simulink model "RobustFormationControl_FractionalModel"  (R2023a)
settings: Solver=ode3  StartTime=0.0  StopTime=30  FixedStep=0.0001  RelTol=1e-3
InitFcn:
  | % close all;
  | % clear all;
  | % clc;
  | % System & Qaudrotor Parameters
  | %==============================
  | m = 0.486;                                         % Quadrotor Mass ( kg )
  | 
  | L = 0.25;                                         % Length of the arm ( m )
  | % L = 0.25;                                         % Length of the arm ( m )
  | 
  | Ixx = 4.856e-03; Iyy = 4.856e-03; Izz = 8.801e-03; % The moments of inertia around x,y and z axes respectively ( kg.m^2 )
  | % Ixx = 3.8278e-03; Iyy = 3.8278e-03; Izz = 7.6566e-03; % The moments of inertia around x,y and z axes respectively ( kg.m^2 )
  | 
  | Jr = 2.8385e-5;                                            % The inertia moment of rotor ( kg.m^2 )
  | % Jr = 0;
  | 
  | % Kx=5.5670e-4;
  | % Ky=5.5670e-4;
  | % Kz=6.3540e-4;
  | % kx=0.032;
  | % ky=0.032;
  | % kz=0.048;
  | Kfx = 5.5670e-4; Kfy = 5.5670e-4; Kfz = 6.3540e-4;% The Rotational drag cofficients ( N/rad/s )
  | 
  | % Ktx = 0.032; Kty = 0.032; Ktz = 0.048;               % The linear drag coefficients in x, y, z respectively ( N/m/s )
  | Ktx = 5.5670e-4; Kty =5.5670e-4; Ktz = 6.3540e-4;               % The linear drag coefficients in x, y, z respectively ( N/m/s )
  | 
  | b = 2.923e-05;                                      % The lift coefficient
  | % b = 2.9842e-05;                                      % The lift coefficient
  | 
  | d = 1.12e-06;                                       % The drag coefficient
  | % d = 3.2320e-07;                                       % The drag coefficient
  | 
  | g = 9.81;                                          % The acceleration due to gravity ( m/s^2 )
  | 
  | %-------- The Coefficients of Non-linear Equations of Quadrotor ( Page 11) -------
  | %--------------------------------------------------------------------------------
  | % Rotational Equations
  | %=====================
  | % Coefficients in ( eq1 ) >>..
  | a1 = (Iyy - Izz)/Ixx;
  | b1 = - Jr/Ixx;
  | c1 = - Kfx/Ixx;
  | d1 = L/Ixx;
  | 
  | % Coefficients in ( eq2 ) >>..
  | a2 = (Izz - Ixx)/Iyy;
  | b2 = Jr/Iyy;
  | c2 = - Kfy/Iyy;
  | d2 = L/Iyy;
  | 
  | % Coefficients in ( eq3 ) >>..
  | a3 = (Ixx - Iyy)/Izz;
  | b3 = - Kfz/Izz;
  | c3 = 1/Izz;
  | % c3 = d/Izz;
  | 
  | % Translational Equations
  | %========================
  | % Coefficients in ( eq4 ) >>..
  | ... (+151 lines)
libraries: fod x135, eeStairGenerator x5
(part 8 of 9)

== system RobustFormationControl_FractionalModel/Fractional Leader with four followers/Follower 3 System/Follower 2 Quadrotor Model/Control Module1/Subsystem6/Subsystem4 ==
  x8 : Inport
  xL : Inport  Port=2
  dX : Inport  Port=3
  Derivative{,1..3} (4 alike) : Derivative
  Divide2 : Product  Inputs=**  RndMeth=Zero  SaturateOnIntegerOverflow=on
  Gain1 : Gain  Commented=on  Gain=a6
  Sum : Sum  Inputs=-+-
  D1 : Outport
  wires:
  Sum/1 -> D1/1
  x8/1 -> Divide2/2
  Divide2/1 -> Sum/1
  [a4D] -> Divide2/1
  Derivative/1 -> Derivative1/1
  xL/1 -> Derivative/1
  Derivative3/1 -> Sum/3
  Derivative2/1 -> Derivative3/1
  dX/1 -> Derivative2/1
  Derivative1/1 -> Sum/2

== system RobustFormationControl_FractionalModel/Fractional Leader with four followers/Follower 3 System/Follower 2 Quadrotor Model/Control Module1/Subsystem6/Subsystem5 ==
  xL : Inport
  x7 : Inport  Port=2
  x8 : Inport  Port=3
  dX : Inport  Port=4
  S8 : Inport  Port=5
  Abs : Abs  SaturateOnIntegerOverflow=off
  Derivative : Derivative
  Derivative1 : Derivative
  Divide{,1..4} (5 alike) : Product  Inputs=**  RndMeth=Zero  SaturateOnIntegerOverflow=on
  Gain : Gain  Gain=q0
  Gain1 : Gain  Gain=q1
  Gain2 : Gain  Gain=q2
  Integrator : Integrator
  Integrator1 : Integrator
  Integrator2 : Integrator
  Sum2 : Sum  Inputs=++++
  Sum4 : Sum  Inputs=+--
  Sum5 : Sum  Inputs=+--
  Tanh : Trigonometry  Operator=tanh
  w : Constant  Value=w
  D3 : Outport  VectorParamsAs1DForOutWhenUnconnected=off
  wires:
  S8/1 -> [S8], Abs/1
  Gain/1 -> Integrator/1
  Integrator/1 -> Sum2/1  "B0"
  [e1] -> Divide/2
  Gain1/1 -> Integrator1/1
  Divide/1 -> Gain1/1
  Divide1/1 -> Gain2/1
  Gain2/1 -> Integrator2/1
  [e2] -> Divide1/2
  Abs/1 -> Divide1/1, Divide/1, Gain/1
  Integrator1/1 -> Divide3/2  "B1"
  w/1 -> Sum2/4
  Tanh/1 -> Divide2/2
  [S8] -> Tanh/1
  Divide2/1 -> D3/1
  [e1] -> Divide3/1
  [e2] -> Divide4/1
  Integrator2/1 -> Divide4/2  "B2"
  Divide3/1 -> Sum2/2
  Divide4/1 -> Sum2/3
  Sum2/1 -> Divide2/1
  Derivative1/1 -> Sum4/3
  Derivative/1 -> Sum4/1
  Sum4/1 -> [e2]
  Sum5/1 -> [e1]
  xL/1 -> Sum5/1, Derivative/1
  x8/1 -> Sum4/2
  dX/1 -> Sum5/3, Derivative1/1
  x7/1 -> Sum5/2

== system RobustFormationControl_FractionalModel/Fractional Leader with four followers/Follower 3 System/Follower 2 Quadrotor Model/Control Module1/Subsystem8/Subsystem ==
  x3 : Inport
  xd3 : Inport  Port=2
  x4 : Inport  Port=3
  xd4 : Inport  Port=4
  S4 : Inport  Port=5
  Constant : Constant  Value=p/q
  Constant1 : Constant  Value=gammaP(2)-1
  Divide : Product  Inputs=**  RndMeth=Zero  SaturateOnIntegerOverflow=on
  Fractional derivative : fod/Fractional derivative  gam=alpha1(2)  ww=[0.001; 1000]  n=5  nFod=off
      settings: SourceProductName=FOMCON Toolbox
  Fractional integrator1 : fod/Fractional integrator  gam=alpha2(2)  ww=[0.001; 1000]  n=5  nFod=off
      settings: SourceProductName=FOMCON Toolbox
  Gain : Gain  Gain=cTheta1
  Gain1 : Gain  Gain=cTheta2
  Gain2 : Gain  Gain=gammaP(2)
  Gain3 : Gain  Gain=Sigma1Theta
  Gain4 : Gain  Gain=Sigma2Theta
  Power : Math  Operator=pow
  Power1 : Math  Operator=pow
  Sum : Sum
  Sum1 : Sum  Inputs=+-
  Sum2 : Sum  Inputs=---
  Sum3 : Sum  Inputs=+-
  Tanh : Trigonometry  Operator=tanh
  D2 : Outport  VectorParamsAs1DForOutWhenUnconnected=off
  wires:
  xd4/1 -> Sum1/2
  xd3/1 -> Sum3/2
  x3/1 -> Sum3/1
  x4/1 -> Sum1/1
  Sum3/1 -> Power1/1, Power/1
  Constant/1 -> Power/2
  Power/1 -> Gain/1
  Gain/1 -> Fractional derivative/1
  Constant1/1 -> Power1/2
  Power1/1 -> Divide/2
  Divide/1 -> Gain1/1
  Gain1/1 -> Gain2/1
  Sum1/1 -> Divide/1
  Gain2/1 -> Fractional integrator1/1
  S4/1 -> Tanh/1, Gain4/1
  Tanh/1 -> Gain3/1
  Gain3/1 -> Sum/1
  Gain4/1 -> Sum/2
  Sum/1 -> Sum2/3
  Fractional derivative/1 -> Sum2/1
  Fractional integrator1/1 -> Sum2/2
  Sum2/1 -> D2/1

== system RobustFormationControl_FractionalModel/Fractional Leader with four followers/Follower 3 System/Follower 2 Quadrotor Model/Control Module1/Subsystem8/Subsystem1 ==
  x4 : Inport
  x6 : Inport  Port=2
  x2 : Inport  Port=3
  Omega : Inport  Port=4
  xd4 : Inport  Port=5
  Gain1 : Gain  Gain=a2
  Gain2 : Gain  Gain=c2
  Gain3 : Gain  Gain=b2
  Math Function1 : Math  Operator=square  SignedPower=on
  Product2 : Product
  Product4 : Product
  Sum3 : Sum  Inputs=---+
  D1 : Outport
  wires:
  x6/1 -> Product2/2
  Gain1/1 -> Sum3/1  "a1 x4 x6"
  Sum3/1 -> D1/1
  Math Function1/1 -> Gain2/1  "x2^2"
  x2/1 -> Product4/1, Product2/1
  x4/1 -> Math Function1/1
  xd4/1 -> Sum3/4
  Product4/1 -> Gain3/1
  Omega/1 -> Product4/2
  Product2/1 -> Gain1/1
  Gain3/1 -> Sum3/3
  Gain2/1 -> Sum3/2  "c1 x2^2"

== system RobustFormationControl_FractionalModel/Fractional Leader with four followers/Follower 3 System/Follower 2 Quadrotor Model/Control Module1/Subsystem8/Subsystem2 ==
  x3 : Inport
  xd3 : Inport  Port=2
  x4 : Inport  Port=3
  xd4 : Inport  Port=4
  S4 : Inport  Port=5
  Abs : Abs  SaturateOnIntegerOverflow=off
  Divide{,1..4} (5 alike) : Product  Inputs=**  RndMeth=Zero  SaturateOnIntegerOverflow=on
  Gain : Gain  Gain=q0
  Gain1 : Gain  Gain=q1
  Gain2 : Gain  Gain=q2
  Integrator : Integrator
  Integrator1 : Integrator
  Integrator2 : Integrator
  Sum1 : Sum  Inputs=+-
  Sum2 : Sum  Inputs=----
  Sum3 : Sum  Inputs=+-
  Tanh : Trigonometry  Operator=tanh
  w : Constant  Value=w
  D3 : Outport  VectorParamsAs1DForOutWhenUnconnected=off
  wires:
  xd4/1 -> Sum1/2
  xd3/1 -> Sum3/2
  x3/1 -> Sum3/1
  x4/1 -> Sum1/1
  S4/1 -> [S4], Abs/1
  Sum1/1 -> [e2]
  Sum3/1 -> [e1]
  Gain/1 -> Integrator/1
  Integrator/1 -> Sum2/1  "B0"
  [e1] -> Divide/2
  Gain1/1 -> Integrator1/1
  Divide/1 -> Gain1/1
  Divide1/1 -> Gain2/1
  Gain2/1 -> Integrator2/1
  [e2] -> Divide1/2
  Abs/1 -> Divide1/1, Divide/1, Gain/1
  Integrator1/1 -> Divide3/2  "B1"
  w/1 -> Sum2/4
  Tanh/1 -> Divide2/2
  [S4] -> Tanh/1
  Divide2/1 -> D3/1
  [e1] -> Divide3/1
  [e2] -> Divide4/1
  Integrator2/1 -> Divide4/2  "B2"
  Divide3/1 -> Sum2/2
  Divide4/1 -> Sum2/3
  Sum2/1 -> Divide2/1

== system RobustFormationControl_FractionalModel/Fractional Leader with four followers/Follower 3 System/Follower 2 Quadrotor Model/Quadrotor Dynamic System/Rotational System/Equation1 ==
  x4 : Inport
  x6 : Inport  Port=2
  U2 : Inport  Port=3
  Omega : Inport  Port=4
  Gain : Gain  Gain=a1
  Gain1 : Gain  Gain=c1
  Gain2 : Gain  Gain=b1
  Gain3 : Gain  Gain=d1
  Integrator : Integrator
  Integrator1 : Integrator
  Math Function : Math  Operator=square  SignedPower=on
  Product : Product
  Product1 : Product
  Sum : Sum  Inputs=|++++
  x1 = Phi : Outport  VectorParamsAs1DForOutWhenUnconnected=off
  x2 : Outport  Port=2  VectorParamsAs1DForOutWhenUnconnected=off
  wires:
  Omega/1 -> Product1/2
  Sum/1 -> Integrator/1
  x6/1 -> Product/2
  Product/1 -> Gain/1
  Integrator1/1 -> x1 = Phi/1
  Gain1/1 -> Sum/2  "c1 x2^2"
  Product1/1 -> Gain2/1
  Gain/1 -> Sum/1  "a1 x4 x6"
  Gain3/1 -> Sum/4
  Gain2/1 -> Sum/3
  U2/1 -> Gain3/1
  Integrator/1 -> Integrator1/1, x2/1, Math Function/1
  x4/1 -> Product/1, Product1/1
  Math Function/1 -> Gain1/1  "x2^2"

== system RobustFormationControl_FractionalModel/Fractional Leader with four followers/Follower 3 System/Follower 2 Quadrotor Model/Quadrotor Dynamic System/Rotational System/Equation2 ==
  x2 : Inport
  x6 : Inport  Port=2
  U3 : Inport  Port=3
  Omega : Inport  Port=4
  Gain : Gain  Gain=a2
  Gain1 : Gain  Gain=c2
  Gain2 : Gain  Gain=b2
  Gain3 : Gain  Gain=d2
  Integrator : Integrator
  Integrator1 : Integrator
  Math Function : Math  Operator=square  SignedPower=on
  Product : Product
  Product1 : Product
  Sum : Sum  Inputs=|++++
  x3 =Theta : Outport  VectorParamsAs1DForOutWhenUnconnected=off
  x4 : Outport  Port=2  VectorParamsAs1DForOutWhenUnconnected=off
  wires:
  Omega/1 -> Product1/2
  Sum/1 -> Integrator/1
  x6/1 -> Product/2
  Product/1 -> Gain/1
  Integrator1/1 -> x3 =Theta/1
  Gain1/1 -> Sum/2  "c2 x2^2"
  Product1/1 -> Gain2/1
  Gain/1 -> Sum/1  "a2 x2 x6"
  Gain3/1 -> Sum/4
  Gain2/1 -> Sum/3
  U3/1 -> Gain3/1
  Integrator/1 -> Integrator1/1, x4/1, Math Function/1
  x2/1 -> Product/1, Product1/1
  Math Function/1 -> Gain1/1  "x4^2"

== system RobustFormationControl_FractionalModel/Fractional Leader with four followers/Follower 3 System/Follower 2 Quadrotor Model/Quadrotor Dynamic System/Rotational System/Equation3 ==
  x2 : Inport
  x4 : Inport  Port=2
  U4 : Inport  Port=3
  Gain : Gain  Gain=a3
  Gain1 : Gain  Gain=b3
  Gain3 : Gain  Gain=c3
  Integrator : Integrator
  Integrator1 : Integrator
  Math Function : Math  Operator=square  SignedPower=on
  Product : Product
  Sum : Sum  Inputs=|+++
  x5 =Psi : Outport  VectorParamsAs1DForOutWhenUnconnected=off
  x6 : Outport  Port=2  VectorParamsAs1DForOutWhenUnconnected=off
  wires:
  Sum/1 -> Integrator/1
  x4/1 -> Product/2
  Product/1 -> Gain/1
  Integrator1/1 -> x5 =Psi/1
  Gain1/1 -> Sum/2  "b3 x6^2"
  Gain/1 -> Sum/1  "a3 x2 x4"
  Gain3/1 -> Sum/3
  U4/1 -> Gain3/1
  Integrator/1 -> Integrator1/1, x6/1, Math Function/1
  x2/1 -> Product/1
  Math Function/1 -> Gain1/1  "x6^2"

== system RobustFormationControl_FractionalModel/Fractional Leader with four followers/Follower 3 System/Follower 2 Quadrotor Model/Quadrotor Dynamic System/Translational System/Equation4 ==
  U1 : Inport
  Ux : Inport  Port=2
  Gain : Gain  Gain=1/m
  Gain1 : Gain  Gain=a4
  Integrator : Integrator
  Integrator1 : Integrator  InitialCondition=4
  Product : Product
  Sum : Sum  Inputs=|++
  x7 = x : Outport  VectorParamsAs1DForOutWhenUnconnected=off
  x8 = xdot : Outport  Port=2  VectorParamsAs1DForOutWhenUnconnected=off
  wires:
  Sum/1 -> Integrator/1
  Ux/1 -> Product/2
  Product/1 -> Gain/1
  Integrator1/1 -> x7 = x/1
  Gain1/1 -> Sum/2  "a4 x8"
  Gain/1 -> Sum/1  "U1 Ux / m"
  U1/1 -> Product/1
  Integrator/1 -> Integrator1/1, x8 = xdot/1, Gain1/1

== system RobustFormationControl_FractionalModel/Fractional Leader with four followers/Follower 3 System/Follower 2 Quadrotor Model/Quadrotor Dynamic System/Translational System/Equation5 ==
  U1 : Inport
  Uy : Inport  Port=2
  Gain : Gain  Gain=1/m
  Gain1 : Gain  Gain=a5
  Integrator : Integrator
  Integrator1 : Integrator  InitialCondition=-4
  Product : Product
  Sum : Sum  Inputs=|++
  x9 = y : Outport  VectorParamsAs1DForOutWhenUnconnected=off
  x10 = ydot : Outport  Port=2  VectorParamsAs1DForOutWhenUnconnected=off
  wires:
  Sum/1 -> Integrator/1
  Uy/1 -> Product/2
  Product/1 -> Gain/1
  Integrator1/1 -> x9 = y/1
  Gain1/1 -> Sum/2  "a4 x10"
  Gain/1 -> Sum/1  "U1 Ux / m"
  U1/1 -> Product/1
  Integrator/1 -> Gain1/1, Integrator1/1, x10 = ydot/1

== system RobustFormationControl_FractionalModel/Fractional Leader with four followers/Follower 3 System/Follower 2 Quadrotor Model/Quadrotor Dynamic System/Translational System/Equation6 ==
  U1 : Inport
  x1 : Inport  Port=2
  x3 : Inport  Port=3
  Constant : Constant  Value=g
  Gain : Gain  Gain=1/m
  Gain1 : Gain  Gain=a6
  Integrator : Integrator
  Integrator1 : Integrator
  Product : Product
  Product1 : Product
  Sum : Sum  Inputs=|++-
  Trigonometric Function : Trigonometry  Operator=cos
  Trigonometric Function1 : Trigonometry  Operator=cos
  x11 = z : Outport  VectorParamsAs1DForOutWhenUnconnected=off
  x12 = zdot : Outport  Port=2  VectorParamsAs1DForOutWhenUnconnected=off
  wires:
  Integrator/1 -> Integrator1/1, x12 = zdot/1, Gain1/1
  Constant/1 -> Sum/3
  x3/1 -> Trigonometric Function1/1
  x1/1 -> Trigonometric Function/1
  Trigonometric Function1/1 -> Product1/2
  Trigonometric Function/1 -> Product1/1
  Product1/1 -> Product/2
  Sum/1 -> Integrator/1
  Product/1 -> Gain/1
  Integrator1/1 -> x11 = z/1
  Gain1/1 -> Sum/2  "a6 x12"
  Gain/1 -> Sum/1  "U1 cx1 cx3  / m"
  U1/1 -> Product/1

== system RobustFormationControl_FractionalModel/Fractional Leader with four followers/Follower 4 System/Follower 2 Quadrotor Model/Control Module1/Omega Equations/Control Inputs ==
  w1_sqt : Inport
  w2_sqt : Inport  Port=2
  w3_sqt : Inport  Port=3
  w4_sqt : Inport  Port=4
  Add4 : Sum  Inputs=+-+-
  Omega : Outport  VectorParamsAs1DForOutWhenUnconnected=off
  wires:
  Add4/1 -> Omega/1
  w1_sqt/1 -> Add4/1
  w2_sqt/1 -> Add4/2
  w3_sqt/1 -> Add4/3
  w4_sqt/1 -> Add4/4

== system RobustFormationControl_FractionalModel/Fractional Leader with four followers/Follower 4 System/Follower 2 Quadrotor Model/Control Module1/Subsystem/Subsystem ==
  Ux : Inport
  Uy : Inport  Port=2
  Psi_d : Inport  Port=3
  Product : Product
  Product1 : Product
  Subtract : Sum  Inputs=+-
  Trigonometric Function : Trigonometry
  Trigonometric Function1 : Trigonometry  Operator=cos
  Trigonometric Function2 : Trigonometry  Operator=asin
  Phi_d : Outport  VectorParamsAs1DForOutWhenUnconnected=off
  wires:
  Product1/1 -> Subtract/2
  Uy/1 -> Product1/2
  Ux/1 -> Product/1
  Trigonometric Function1/1 -> Product1/1
  Psi_d/1 -> Trigonometric Function1/1, Trigonometric Function/1
  Product/1 -> Subtract/1
  Subtract/1 -> Trigonometric Function2/1
  Trigonometric Function/1 -> Product/2
  Trigonometric Function2/1 -> Phi_d/1

== system RobustFormationControl_FractionalModel/Fractional Leader with four followers/Follower 4 System/Follower 2 Quadrotor Model/Control Module1/Subsystem/Subsystem1 ==
  Ux : Inport
  Uy : Inport  Port=2
  Psi_d : Inport  Port=3
  Phi_d : Inport  Port=4
  Constant : Constant
  Divide : Product  Inputs=*/
  Product : Product
  Product1 : Product
  Product2 : Product
  Subtract : Sum
  Trigonometric Function : Trigonometry  Operator=cos
  Trigonometric Function1 : Trigonometry
  Trigonometric Function2 : Trigonometry  Operator=asin
  Trigonometric Function3 : Trigonometry  Operator=cos
  Theta_d : Outport  VectorParamsAs1DForOutWhenUnconnected=off
  wires:
  Product1/1 -> Subtract/2
  Uy/1 -> Product1/2
  Ux/1 -> Product/1
  Trigonometric Function1/1 -> Product1/1
  Psi_d/1 -> Trigonometric Function1/1, Trigonometric Function/1
  Product/1 -> Subtract/1
  Trigonometric Function/1 -> Product/2
  Trigonometric Function2/1 -> Theta_d/1
  Constant/1 -> Divide/1
  Product2/1 -> Trigonometric Function2/1
  Subtract/1 -> Product2/1
  Divide/1 -> Product2/2
  Trigonometric Function3/1 -> Divide/2
  Phi_d/1 -> Trigonometric Function3/1

== system RobustFormationControl_FractionalModel/Fractional Leader with four followers/Follower 4 System/Follower 2 Quadrotor Model/Control Module1/Subsystem1/Subsystem ==
  x1 : Inport
  xd1 : Inport  Port=2
  x2 : Inport  Port=3
  xd2 : Inport  Port=4
  Constant : Constant  Value=p/q
  Constant1 : Constant  Value=gx
  Divide : Product  Inputs=**  RndMeth=Zero  SaturateOnIntegerOverflow=on
  Fractional integrator : fod/Fractional integrator  gam=alpha1(1)  ww=[0.001; 1000]  n=5  nFod=off
      settings: SourceProductName=FOMCON Toolbox
  Fractional integrator1 : fod/Fractional integrator  gam=alpha2(1)  ww=[0.001; 1000]  n=5  nFod=off
      settings: SourceProductName=FOMCON Toolbox
  Gain : Gain  Gain=cPhi1
  Gain1 : Gain  Gain=cPhi2
  Power : Math  Operator=pow
  Power1 : Math  Operator=pow
  Sum1 : Sum  Inputs=+-
  Sum2 : Sum  Inputs=+++
  Sum3 : Sum  Inputs=+-
  Tanh : Trigonometry  Operator=tanh
  S2 : Outport  VectorParamsAs1DForOutWhenUnconnected=off
  wires:
  xd2/1 -> Sum1/2
  Sum2/1 -> S2/1
  xd1/1 -> Sum3/2
  x1/1 -> Sum3/1
  x2/1 -> Sum1/1
  Sum3/1 -> Tanh/1, Power1/1, Power/1
  Constant/1 -> Power/2
  Power/1 -> Gain/1
  Gain/1 -> Fractional integrator/1
  Constant1/1 -> Power1/2
  Tanh/1 -> Divide/1
  Power1/1 -> Divide/2
  Divide/1 -> Gain1/1
  Gain1/1 -> Fractional integrator1/1
  Sum1/1 -> Sum2/1
  Fractional integrator/1 -> Sum2/2
  Fractional integrator1/1 -> Sum2/3

== system RobustFormationControl_FractionalModel/Fractional Leader with four followers/Follower 4 System/Follower 2 Quadrotor Model/Control Module1/Subsystem1/Subsystem1 ==
  x5 : Inport
  xd5 : Inport  Port=2
  x6 : Inport  Port=3
  xd6 : Inport  Port=4
  Constant : Constant  Value=p/q
  Constant1 : Constant  Value=gz
  Divide : Product  Inputs=**  RndMeth=Zero  SaturateOnIntegerOverflow=on
  Fractional integrator : fod/Fractional integrator  gam=alpha1(3)  ww=[0.001; 1000]  n=5  nFod=off
      settings: SourceProductName=FOMCON Toolbox
  Fractional integrator1 : fod/Fractional integrator  gam=alpha2(3)  ww=[0.001; 1000]  n=5  nFod=off
      settings: SourceProductName=FOMCON Toolbox
  Gain : Gain  Gain=cPsi1
  Gain1 : Gain  Gain=cPsi2
  Power : Math  Operator=pow
  Power1 : Math  Operator=pow
  Sum1 : Sum  Inputs=+-
  Sum2 : Sum  Inputs=+++
  Sum3 : Sum  Inputs=+-
  Tanh : Trigonometry  Operator=tanh
  S6 : Outport  VectorParamsAs1DForOutWhenUnconnected=off
  wires:
  xd6/1 -> Sum1/2
  Sum2/1 -> S6/1
  xd5/1 -> Sum3/2
  x5/1 -> Sum3/1
  x6/1 -> Sum1/1
  Sum3/1 -> Tanh/1, Power1/1, Power/1
  Constant/1 -> Power/2
  Power/1 -> Gain/1
  Gain/1 -> Fractional integrator/1
  Constant1/1 -> Power1/2
  Tanh/1 -> Divide/1
  Power1/1 -> Divide/2
  Divide/1 -> Gain1/1
  Gain1/1 -> Fractional integrator1/1
  Sum1/1 -> Sum2/1
  Fractional integrator/1 -> Sum2/2
  Fractional integrator1/1 -> Sum2/3

== system RobustFormationControl_FractionalModel/Fractional Leader with four followers/Follower 4 System/Follower 2 Quadrotor Model/Control Module1/Subsystem1/Subsystem2 ==
  yL : Inport
  x9 : Inport  Port=2
  x10 : Inport  Port=3
  dY : Inport  Port=4
  Constant : Constant  Value=p/q
  Constant1 : Constant  Value=gy
  Derivative : Derivative
  Derivative1 : Derivative
  Divide : Product  Inputs=**  RndMeth=Zero  SaturateOnIntegerOverflow=on
  Fractional integrator : fod/Fractional integrator  gam=alpha1(2)  ww=[0.001; 1000]  n=5  nFod=off
      settings: SourceProductName=FOMCON Toolbox
  Fractional integrator1 : fod/Fractional integrator  gam=alpha2(2)  ww=[0.001; 1000]  n=5  nFod=off
      settings: SourceProductName=FOMCON Toolbox
  Gain2 : Gain  Gain=cy1
  Gain3 : Gain  Gain=cy2
  Power : Math  Operator=pow
  Power1 : Math  Operator=pow
  Sum1 : Sum  Inputs=+--
  Sum3 : Sum  Inputs=+--
  Sum5 : Sum  Inputs=+++
  Tanh : Trigonometry  Operator=tanh
  S10 : Outport  VectorParamsAs1DForOutWhenUnconnected=off
  wires:
  x9/1 -> Sum3/2
  yL/1 -> Sum3/1, Derivative/1
  dY/1 -> Sum3/3, Derivative1/1
  x10/1 -> Sum1/3
  Derivative/1 -> Sum1/1
  Derivative1/1 -> Sum1/2
  Fractional integrator1/1 -> Sum5/3
  Fractional integrator/1 -> Sum5/2
  Gain3/1 -> Fractional integrator1/1
  Sum1/1 -> Sum5/1
  Sum5/1 -> S10/1
  Divide/1 -> Gain3/1
  Gain2/1 -> Fractional integrator/1
  Tanh/1 -> Divide/1
  Power1/1 -> Divide/2
  Power/1 -> Gain2/1
  Constant1/1 -> Power1/2
  Sum3/1 -> Tanh/1, Power1/1, Power/1
  Constant/1 -> Power/2

== system RobustFormationControl_FractionalModel/Fractional Leader with four followers/Follower 4 System/Follower 2 Quadrotor Model/Control Module1/Subsystem1/Subsystem3 ==
  xL : Inport
  x7 : Inport  Port=2
  x8 : Inport  Port=3
  dX : Inport  Port=4
  Constant : Constant  Value=p/q
  Constant1 : Constant  Value=gx
  Derivative : Derivative
  Derivative1 : Derivative
  Divide : Product  Inputs=**  RndMeth=Zero  SaturateOnIntegerOverflow=on
  Fractional integrator : fod/Fractional integrator  gam=alpha1(1)  ww=[0.001; 1000]  n=5  nFod=off
      settings: SourceProductName=FOMCON Toolbox
  Fractional integrator1 : fod/Fractional integrator  gam=alpha2(1)  ww=[0.001; 1000]  n=5  nFod=off
      settings: SourceProductName=FOMCON Toolbox
  Gain2 : Gain  Gain=cx1
  Gain3 : Gain  Gain=cx2
  Power : Math  Operator=pow
  Power1 : Math  Operator=pow
  Sum1 : Sum  Inputs=+--
  Sum3 : Sum  Inputs=+--
  Sum5 : Sum  Inputs=+++
  Tanh : Trigonometry  Operator=tanh
  S8 : Outport  VectorParamsAs1DForOutWhenUnconnected=off
  wires:
  x7/1 -> Sum3/2
  xL/1 -> Sum3/1, Derivative/1
  dX/1 -> Sum3/3, Derivative1/1
  x8/1 -> Sum1/3
  Derivative/1 -> Sum1/1
  Derivative1/1 -> Sum1/2
  Fractional integrator1/1 -> Sum5/3
  Fractional integrator/1 -> Sum5/2
  Gain3/1 -> Fractional integrator1/1
  Sum1/1 -> Sum5/1
  Sum5/1 -> S8/1
  Divide/1 -> Gain3/1
  Gain2/1 -> Fractional integrator/1
  Tanh/1 -> Divide/1
  Power1/1 -> Divide/2
  Power/1 -> Gain2/1
  Constant1/1 -> Power1/2
  Sum3/1 -> Tanh/1, Power1/1, Power/1
  Constant/1 -> Power/2

== system RobustFormationControl_FractionalModel/Fractional Leader with four followers/Follower 4 System/Follower 2 Quadrotor Model/Control Module1/Subsystem1/Subsystem4 ==
  zL : Inport
  x11 : Inport  Port=2
  x12 : Inport  Port=3
  dZ : Inport  Port=4
  Constant : Constant  Value=p/q
  Constant1 : Constant  Value=gz
  Derivative : Derivative
  Derivative1 : Derivative
  Divide : Product  Inputs=**  RndMeth=Zero  SaturateOnIntegerOverflow=on
  Fractional integrator : fod/Fractional integrator  gam=alpha1(2)  ww=[0.001; 1000]  n=5  nFod=off
      settings: SourceProductName=FOMCON Toolbox
  Fractional integrator1 : fod/Fractional integrator  gam=alpha2(2)  ww=[0.001; 1000]  n=5  nFod=off
      settings: SourceProductName=FOMCON Toolbox
  Gain2 : Gain  Gain=cz1
  Gain3 : Gain  Gain=cz2
  Power : Math  Operator=pow
  Power1 : Math  Operator=pow
  Sum1 : Sum  Inputs=+--
  Sum3 : Sum  Inputs=+--
  Sum5 : Sum  Inputs=+++
  Tanh : Trigonometry  Operator=tanh
  S12 : Outport  VectorParamsAs1DForOutWhenUnconnected=off
  wires:
  Constant/1 -> Power/2
  Sum3/1 -> Power/1, Tanh/1, Power1/1
  Constant1/1 -> Power1/2
  Power/1 -> Gain2/1
  Power1/1 -> Divide/2
  Tanh/1 -> Divide/1
  Gain2/1 -> Fractional integrator/1
  Divide/1 -> Gain3/1
  Sum5/1 -> S12/1
  Sum1/1 -> Sum5/1
  Gain3/1 -> Fractional integrator1/1
  Fractional integrator/1 -> Sum5/2
  Fractional integrator1/1 -> Sum5/3
  Derivative1/1 -> Sum1/2
  Derivative/1 -> Sum1/1
  x12/1 -> Sum1/3
  dZ/1 -> Derivative1/1, Sum3/3
  zL/1 -> Derivative/1, Sum3/1
  x11/1 -> Sum3/2

== system RobustFormationControl_FractionalModel/Fractional Leader with four followers/Follower 4 System/Follower 2 Quadrotor Model/Control Module1/Subsystem1/Subsystem6 ==
  x3 : Inport
  xd3 : Inport  Port=2
  x4 : Inport  Port=3
  xd4 : Inport  Port=4
  Constant : Constant  Value=p/q
  Constant1 : Constant  Value=gy
  Divide : Product  Inputs=**  RndMeth=Zero  SaturateOnIntegerOverflow=on
  Fractional integrator : fod/Fractional integrator  gam=alpha1(2)  ww=[0.001; 1000]  n=5  nFod=off
      settings: SourceProductName=FOMCON Toolbox
  Fractional integrator1 : fod/Fractional integrator  gam=alpha2(2)  ww=[0.001; 1000]  n=5  nFod=off
      settings: SourceProductName=FOMCON Toolbox
  Gain : Gain  Gain=cTheta1
  Gain1 : Gain  Gain=cTheta2
  Power : Math  Operator=pow
  Power1 : Math  Operator=pow
  Sum1 : Sum  Inputs=+-
  Sum2 : Sum  Inputs=+++
  Sum3 : Sum  Inputs=+-
  Tanh : Trigonometry  Operator=tanh
  S4 : Outport  VectorParamsAs1DForOutWhenUnconnected=off
  wires:
  xd4/1 -> Sum1/2
  Sum2/1 -> S4/1
  xd3/1 -> Sum3/2
  x3/1 -> Sum3/1
  x4/1 -> Sum1/1
  Sum3/1 -> Tanh/1, Power1/1, Power/1
  Constant/1 -> Power/2
  Power/1 -> Gain/1
  Gain/1 -> Fractional integrator/1
  Constant1/1 -> Power1/2
  Tanh/1 -> Divide/1
  Power1/1 -> Divide/2
  Divide/1 -> Gain1/1
  Gain1/1 -> Fractional integrator1/1
  Sum1/1 -> Sum2/1
  Fractional integrator/1 -> Sum2/2
  Fractional integrator1/1 -> Sum2/3

== system RobustFormationControl_FractionalModel/Fractional Leader with four followers/Follower 4 System/Follower 2 Quadrotor Model/Control Module1/Subsystem10/Subsystem ==
  zL : Inport
  x11 : Inport  Port=2
  x12 : Inport  Port=3
  dZ : Inport  Port=4
  S12 : Inport  Port=5
  Constant : Constant  Value=p/q
  Constant1 : Constant  Value=gz-1
  Derivative : Derivative
  Derivative1 : Derivative
  Divide : Product  Inputs=**  RndMeth=Zero  SaturateOnIntegerOverflow=on
  Fractional derivative : fod/Fractional derivative  gam=alpha1(3)  ww=[0.001; 1000]  n=5  nFod=off
      settings: SourceProductName=FOMCON Toolbox
  Fractional integrator1 : fod/Fractional integrator  gam=alpha2(3)  ww=[0.001; 1000]  n=5  nFod=off
      settings: SourceProductName=FOMCON Toolbox
  Gain : Gain  Gain=cz1
  Gain1 : Gain  Gain=cz2
  Gain2 : Gain  Gain=gz
  Gain3 : Gain  Gain=Sigma1Z
  Gain4 : Gain  Gain=Sigma2Z
  Power : Math  Operator=pow
  Power1 : Math  Operator=pow
  Sum : Sum
  Sum1 : Sum  Inputs=+--
  Sum2 : Sum  Inputs=+++
  Sum3 : Sum  Inputs=+--
  Tanh : Trigonometry  Operator=tanh
  D2 : Outport  VectorParamsAs1DForOutWhenUnconnected=off
  wires:
  Sum3/1 -> Power1/1, Power/1
  Constant/1 -> Power/2
  Power/1 -> Gain/1
  Gain/1 -> Fractional derivative/1
  Constant1/1 -> Power1/2
  Power1/1 -> Divide/2
  Divide/1 -> Gain1/1
  Gain1/1 -> Gain2/1
  Sum1/1 -> Divide/1
  Gain2/1 -> Fractional integrator1/1
  S12/1 -> Tanh/1, Gain4/1
  Tanh/1 -> Gain3/1
  Gain3/1 -> Sum/1
  Gain4/1 -> Sum/2
  Sum/1 -> Sum2/3
  Fractional derivative/1 -> Sum2/1
  Fractional integrator1/1 -> Sum2/2
  Sum2/1 -> D2/1
  zL/1 -> Sum3/1, Derivative/1
  Derivative/1 -> Sum1/1
  x12/1 -> Sum1/2
  dZ/1 -> Sum3/3, Derivative1/1
  Derivative1/1 -> Sum1/3
  x11/1 -> Sum3/2

== system RobustFormationControl_FractionalModel/Fractional Leader with four followers/Follower 4 System/Follower 2 Quadrotor Model/Control Module1/Subsystem10/Subsystem1 ==
  x12 : Inport
  zL : Inport  Port=2
  dZ : Inport  Port=3
  Constant2 : Constant  Value=g
  Derivative{,1..3} (4 alike) : Derivative
  Divide2 : Product  Inputs=**  RndMeth=Zero  SaturateOnIntegerOverflow=on
  Gain1 : Gain  Commented=on  Gain=a6
  Sum : Sum  Inputs=-++-
  D1 : Outport
  wires:
  Sum/1 -> D1/1
  x12/1 -> Divide2/2
  Divide2/1 -> Sum/1
  Constant2/1 -> Sum/2
  [a6D] -> Divide2/1
  Derivative/1 -> Derivative1/1
  Derivative1/1 -> Sum/3
  zL/1 -> Derivative/1
  Derivative3/1 -> Sum/4
  Derivative2/1 -> Derivative3/1
  dZ/1 -> Derivative2/1

== system RobustFormationControl_FractionalModel/Fractional Leader with four followers/Follower 4 System/Follower 2 Quadrotor Model/Control Module1/Subsystem10/Subsystem2 ==
  zL : Inport
  x11 : Inport  Port=2
  x12 : Inport  Port=3
  dZ : Inport  Port=4
  S12 : Inport  Port=5
  Abs : Abs  SaturateOnIntegerOverflow=off
  Derivative : Derivative
  Derivative1 : Derivative
  Divide{,1..4} (5 alike) : Product  Inputs=**  RndMeth=Zero  SaturateOnIntegerOverflow=on
  Gain : Gain  Gain=q0
  Gain1 : Gain  Gain=q1
  Gain2 : Gain  Gain=q2
  Integrator : Integrator
  Integrator1 : Integrator
  Integrator2 : Integrator
  Sum2 : Sum  Inputs=++++
  Sum4 : Sum  Inputs=+--
  Sum5 : Sum  Inputs=+--
  Tanh : Trigonometry  Operator=tanh
  w : Constant  Value=w
  D3 : Outport  VectorParamsAs1DForOutWhenUnconnected=off
  wires:
  S12/1 -> [S12], Abs/1
  Gain/1 -> Integrator/1
  Integrator/1 -> Sum2/1  "B0"
  [e1] -> Divide/2
  Gain1/1 -> Integrator1/1
  Divide/1 -> Gain1/1
  Divide1/1 -> Gain2/1
  Gain2/1 -> Integrator2/1
  [e2] -> Divide1/2
  Abs/1 -> Divide1/1, Divide/1, Gain/1
  Integrator1/1 -> Divide3/2  "B1"
  w/1 -> Sum2/4
  Tanh/1 -> Divide2/2
  [S12] -> Tanh/1
  Divide2/1 -> D3/1
  [e1] -> Divide3/1
  [e2] -> Divide4/1
  Integrator2/1 -> Divide4/2  "B2"
  Divide3/1 -> Sum2/2
  Divide4/1 -> Sum2/3
  Sum2/1 -> Divide2/1
  Derivative1/1 -> Sum4/3
  Derivative/1 -> Sum4/1
  Sum4/1 -> [e2]
  Sum5/1 -> [e1]
  zL/1 -> Sum5/1, Derivative/1
  x12/1 -> Sum4/2
  dZ/1 -> Sum5/3, Derivative1/1
  x11/1 -> Sum5/2

== system RobustFormationControl_FractionalModel/Fractional Leader with four followers/Follower 4 System/Follower 2 Quadrotor Model/Control Module1/Subsystem2/Subsystem3 ==
  yL : Inport
  x9 : Inport  Port=2
  x10 : Inport  Port=3
  dY : Inport  Port=4
  S10 : Inport  Port=5
  Constant : Constant  Value=p/q
  Constant1 : Constant  Value=gy-1
  Derivative : Derivative
  Derivative1 : Derivative
  Divide : Product  Inputs=**  RndMeth=Zero  SaturateOnIntegerOverflow=on
  Fractional derivative : fod/Fractional derivative  gam=alpha1(2)  ww=[0.001; 1000]  n=5  nFod=off
      settings: SourceProductName=FOMCON Toolbox
  Fractional integrator1 : fod/Fractional integrator  gam=alpha2(2)  ww=[0.001; 1000]  n=5  nFod=off
      settings: SourceProductName=FOMCON Toolbox
  Gain : Gain  Gain=cy1
  Gain1 : Gain  Gain=cy2
  Gain2 : Gain  Gain=gy
  Gain3 : Gain  Gain=Sigma1Y
  Gain4 : Gain  Gain=Sigma2Y
  Power : Math  Operator=pow
  Power1 : Math  Operator=pow
  Sum : Sum
  Sum1 : Sum  Inputs=+--
  Sum2 : Sum  Inputs=+++
  Sum3 : Sum  Inputs=+--
  Tanh : Trigonometry  Operator=tanh
  D2 : Outport  VectorParamsAs1DForOutWhenUnconnected=off
  wires:
  Sum3/1 -> Power1/1, Power/1
  Constant/1 -> Power/2
  Power/1 -> Gain/1
  Gain/1 -> Fractional derivative/1
  Constant1/1 -> Power1/2
  Power1/1 -> Divide/2
  Divide/1 -> Gain1/1
  Gain1/1 -> Gain2/1
  Sum1/1 -> Divide/1
  Gain2/1 -> Fractional integrator1/1
  S10/1 -> Tanh/1, Gain4/1
  Tanh/1 -> Gain3/1
  Gain3/1 -> Sum/1
  Gain4/1 -> Sum/2
  Sum/1 -> Sum2/3
  Fractional derivative/1 -> Sum2/1
  Fractional integrator1/1 -> Sum2/2
  Sum2/1 -> D2/1
  yL/1 -> Sum3/1, Derivative/1
  Derivative/1 -> Sum1/1
  x10/1 -> Sum1/2
  dY/1 -> Sum3/3, Derivative1/1
  Derivative1/1 -> Sum1/3
  x9/1 -> Sum3/2

== system RobustFormationControl_FractionalModel/Fractional Leader with four followers/Follower 4 System/Follower 2 Quadrotor Model/Control Module1/Subsystem2/Subsystem4 ==
  x10 : Inport
  yL : Inport  Port=2
  dY : Inport  Port=3
  Derivative{,1..3} (4 alike) : Derivative
  Divide2 : Product  Inputs=**  RndMeth=Zero  SaturateOnIntegerOverflow=on
  Gain1 : Gain  Commented=on  Gain=a5
  Sum : Sum  Inputs=-+-
  D1 : Outport
  wires:
  Sum/1 -> D1/1
  x10/1 -> Divide2/2
  Divide2/1 -> Sum/1
  [a5D] -> Divide2/1
  Derivative/1 -> Derivative1/1
  yL/1 -> Derivative/1
  Derivative3/1 -> Sum/3
  Derivative2/1 -> Derivative3/1
  dY/1 -> Derivative2/1
  Derivative1/1 -> Sum/2

== system RobustFormationControl_FractionalModel/Fractional Leader with four followers/Follower 4 System/Follower 2 Quadrotor Model/Control Module1/Subsystem2/Subsystem5 ==
  yL : Inport
  x9 : Inport  Port=2
  x10 : Inport  Port=3
  dY : Inport  Port=4
  S10 : Inport  Port=5
  Abs : Abs  SaturateOnIntegerOverflow=off
  Derivative : Derivative
  Derivative1 : Derivative
  Divide{,1..4} (5 alike) : Product  Inputs=**  RndMeth=Zero  SaturateOnIntegerOverflow=on
  Gain : Gain  Gain=q0
  Gain1 : Gain  Gain=q1
  Gain2 : Gain  Gain=q2
  Integrator : Integrator
  Integrator1 : Integrator
  Integrator2 : Integrator
  Sum2 : Sum  Inputs=++++
  Sum4 : Sum  Inputs=+--
  Sum5 : Sum  Inputs=+--
  Tanh : Trigonometry  Operator=tanh
  w : Constant  Value=w
  D3 : Outport  VectorParamsAs1DForOutWhenUnconnected=off
  wires:
  S10/1 -> [S10], Abs/1
  Gain/1 -> Integrator/1
  Integrator/1 -> Sum2/1  "B0"
  [e1] -> Divide/2
  Gain1/1 -> Integrator1/1
  Divide/1 -> Gain1/1
  Divide1/1 -> Gain2/1
  Gain2/1 -> Integrator2/1
  [e2] -> Divide1/2
  Abs/1 -> Divide1/1, Divide/1, Gain/1
  Integrator1/1 -> Divide3/2  "B1"
  w/1 -> Sum2/4
  Tanh/1 -> Divide2/2
  [S10] -> Tanh/1
  Divide2/1 -> D3/1
  [e1] -> Divide3/1
  [e2] -> Divide4/1
  Integrator2/1 -> Divide4/2  "B2"
  Divide3/1 -> Sum2/2
  Divide4/1 -> Sum2/3
  Sum2/1 -> Divide2/1
  Derivative1/1 -> Sum4/3
  Derivative/1 -> Sum4/1
  Sum4/1 -> [e2]
  Sum5/1 -> [e1]
  yL/1 -> Sum5/1, Derivative/1
  x10/1 -> Sum4/2
  dY/1 -> Sum5/3, Derivative1/1
  x9/1 -> Sum5/2

== system RobustFormationControl_FractionalModel/Fractional Leader with four followers/Follower 4 System/Follower 2 Quadrotor Model/Control Module1/Subsystem4/Subsystem ==
  x1 : Inport
  xd1 : Inport  Port=2
  x2 : Inport  Port=3
  xd2 : Inport  Port=4
  S2 : Inport  Port=5
  Constant : Constant  Value=p/q
  Constant1 : Constant  Value=gammaP(1)-1
  Divide : Product  Inputs=**  RndMeth=Zero  SaturateOnIntegerOverflow=on
  Fractional derivative : fod/Fractional derivative  gam=alpha1(1)  ww=[0.001; 1000]  n=5  nFod=off
      settings: SourceProductName=FOMCON Toolbox
  Fractional integrator1 : fod/Fractional integrator  gam=alpha2(2)  ww=[0.001; 1000]  n=5  nFod=off
      settings: SourceProductName=FOMCON Toolbox
  Gain : Gain  Gain=cPhi1
  Gain1 : Gain  Gain=cPhi2
  Gain2 : Gain  Gain=gammaP(1)
  Gain3 : Gain  Gain=Sigma1Phi
  Gain4 : Gain  Gain=Sigma1Phi
  Power : Math  Operator=pow
  Power1 : Math  Operator=pow
  Sum : Sum
  Sum1 : Sum  Inputs=+-
  Sum2 : Sum  Inputs=---
  Sum3 : Sum  Inputs=+-
  Tanh : Trigonometry  Operator=tanh
  D2 : Outport  VectorParamsAs1DForOutWhenUnconnected=off
  wires:
  xd2/1 -> Sum1/2
  xd1/1 -> Sum3/2
  x1/1 -> Sum3/1
  x2/1 -> Sum1/1
  Sum3/1 -> Power1/1, Power/1
  Constant/1 -> Power/2
  Power/1 -> Gain/1
  Gain/1 -> Fractional derivative/1
  Constant1/1 -> Power1/2
  Power1/1 -> Divide/2
  Divide/1 -> Gain1/1
  Gain1/1 -> Gain2/1
  Sum1/1 -> Divide/1
  Gain2/1 -> Fractional integrator1/1
  S2/1 -> Tanh/1, Gain4/1
  Tanh/1 -> Gain3/1
  Gain3/1 -> Sum/1
  Gain4/1 -> Sum/2
  Sum/1 -> Sum2/3
  Fractional derivative/1 -> Sum2/1
  Fractional integrator1/1 -> Sum2/2
  Sum2/1 -> D2/1

== system RobustFormationControl_FractionalModel/Fractional Leader with four followers/Follower 4 System/Follower 2 Quadrotor Model/Control Module1/Subsystem4/Subsystem1 ==
  x4 : Inport
  x6 : Inport  Port=2
  x2 : Inport  Port=3
  Omega : Inport  Port=4
  xd2 : Inport  Port=5
  Gain : Gain  Gain=a1
  Gain6 : Gain  Gain=c1
  Gain7 : Gain  Gain=b1
  Math Function : Math  Operator=square  SignedPower=on
  Product1 : Product
  Product3 : Product
  Sum3 : Sum  Inputs=---+
  D1 : Outport
  wires:
  xd2/1 -> Sum3/4
  Product1/1 -> Gain/1
  Sum3/1 -> D1/1
  Gain6/1 -> Sum3/2  "c1 x2^2"
  Gain7/1 -> Sum3/3
  Product3/1 -> Gain7/1
  Omega/1 -> Product3/2
  Math Function/1 -> Gain6/1  "x2^2"
  x4/1 -> Product3/1, Product1/1
  Gain/1 -> Sum3/1  "a1 x4 x6"
  x6/1 -> Product1/2
  x2/1 -> Math Function/1

== system RobustFormationControl_FractionalModel/Fractional Leader with four followers/Follower 4 System/Follower 2 Quadrotor Model/Control Module1/Subsystem4/Subsystem2 ==
  x1 : Inport
  xd1 : Inport  Port=2
  x2 : Inport  Port=3
  xd2 : Inport  Port=4
  S2 : Inport  Port=5
  Abs : Abs  SaturateOnIntegerOverflow=off
  Divide{,1..4} (5 alike) : Product  Inputs=**  RndMeth=Zero  SaturateOnIntegerOverflow=on
  Gain : Gain  Gain=q0
  Gain1 : Gain  Gain=q1
  Gain2 : Gain  Gain=q2
  Integrator : Integrator
  Integrator1 : Integrator
  Integrator2 : Integrator
  Scope : Scope  NumInputPorts=3
  Sum1 : Sum  Inputs=+-
  Sum2 : Sum  Inputs=----
  Sum3 : Sum  Inputs=+-
  Tanh : Trigonometry  Operator=tanh
  w : Constant  Value=w
  D3 : Outport  VectorParamsAs1DForOutWhenUnconnected=off
  wires:
  xd2/1 -> Sum1/2
  xd1/1 -> Sum3/2
  x1/1 -> Sum3/1
  x2/1 -> Sum1/1
  S2/1 -> [S2], Abs/1
  Sum1/1 -> [e2]
  Sum3/1 -> [e1]
  Gain/1 -> Integrator/1
  Integrator/1 -> Scope/1, Sum2/1  "B0"
  [e1] -> Divide/2
  Gain1/1 -> Integrator1/1
  Divide/1 -> Gain1/1
  Divide1/1 -> Gain2/1
  Gain2/1 -> Integrator2/1
  [e2] -> Divide1/2
  Abs/1 -> Divide1/1, Divide/1, Gain/1
  Integrator1/1 -> Divide3/2, Scope/2  "B1"
  w/1 -> Sum2/4
  Tanh/1 -> Divide2/2
  [S2] -> Tanh/1
  Divide2/1 -> D3/1
  [e1] -> Divide3/1
  [e2] -> Divide4/1
  Integrator2/1 -> Divide4/2, Scope/3  "B2"
  Divide3/1 -> Sum2/2
  Divide4/1 -> Sum2/3
  Sum2/1 -> Divide2/1

== system RobustFormationControl_FractionalModel/Fractional Leader with four followers/Follower 4 System/Follower 2 Quadrotor Model/Control Module1/Subsystem5/Subsystem ==
  x5 : Inport
  xd5 : Inport  Port=2
  x6 : Inport  Port=3
  xd6 : Inport  Port=4
  S4 : Inport  Port=5
  Constant : Constant  Value=p/q
  Constant1 : Constant  Value=gammaP(3)-1
  Divide : Product  Inputs=**  RndMeth=Zero  SaturateOnIntegerOverflow=on
  Fractional derivative : fod/Fractional derivative  gam=alpha1(3)  ww=[0.001; 1000]  n=5  nFod=off
      settings: SourceProductName=FOMCON Toolbox
  Fractional integrator1 : fod/Fractional integrator  gam=alpha2(2)  ww=[0.001; 1000]  n=5  nFod=off
      settings: SourceProductName=FOMCON Toolbox
  Gain : Gain  Gain=cPsi1
  Gain1 : Gain  Gain=cPsi2
  Gain2 : Gain  Gain=gammaP(3)
  Gain3 : Gain  Gain=Sigma1Psi
  Gain4 : Gain  Gain=Sigma2Psi
  Power : Math  Operator=pow
  Power1 : Math  Operator=pow
  Sum : Sum
  Sum1 : Sum  Inputs=+-
  Sum2 : Sum  Inputs=---
  Sum3 : Sum  Inputs=+-
  Tanh : Trigonometry  Operator=tanh
  D2 : Outport  VectorParamsAs1DForOutWhenUnconnected=off
  wires:
  xd6/1 -> Sum1/2
  xd5/1 -> Sum3/2
  x5/1 -> Sum3/1
  x6/1 -> Sum1/1
  Sum3/1 -> Power1/1, Power/1
  Constant/1 -> Power/2
  Power/1 -> Gain/1
  Gain/1 -> Fractional derivative/1
  Constant1/1 -> Power1/2
  Power1/1 -> Divide/2
  Divide/1 -> Gain1/1
  Gain1/1 -> Gain2/1
  Sum1/1 -> Divide/1
  Gain2/1 -> Fractional integrator1/1
  S4/1 -> Tanh/1, Gain4/1
  Tanh/1 -> Gain3/1
  Gain3/1 -> Sum/1
  Gain4/1 -> Sum/2
  Sum/1 -> Sum2/3
  Fractional derivative/1 -> Sum2/1
  Fractional integrator1/1 -> Sum2/2
  Sum2/1 -> D2/1

== system RobustFormationControl_FractionalModel/Fractional Leader with four followers/Follower 4 System/Follower 2 Quadrotor Model/Control Module1/Subsystem5/Subsystem1 ==
  x4 : Inport
  x6 : Inport  Port=2
  x2 : Inport  Port=3
  xd6 : Inport  Port=4
  Gain : Gain  Gain=a3
  Gain6 : Gain  Gain=b3
  Math Function : Math  Operator=square  SignedPower=on
  Product1 : Product
  Sum1 : Sum  Inputs=--+
  D1 : Outport
  wires:
  x6/1 -> Math Function/1
  Product1/1 -> Gain/1
  xd6/1 -> Sum1/3
  Gain6/1 -> Sum1/2  "c1 x2^2"
  Math Function/1 -> Gain6/1  "x2^2"
  x2/1 -> Product1/1
  Gain/1 -> Sum1/1  "a1 x4 x6"
  x4/1 -> Product1/2
  Sum1/1 -> D1/1

== system RobustFormationControl_FractionalModel/Fractional Leader with four followers/Follower 4 System/Follower 2 Quadrotor Model/Control Module1/Subsystem5/Subsystem2 ==
  x5 : Inport
  xd5 : Inport  Port=2
  x6 : Inport  Port=3
  xd6 : Inport  Port=4
  S6 : Inport  Port=5
  Abs : Abs  SaturateOnIntegerOverflow=off
  Divide{,1..4} (5 alike) : Product  Inputs=**  RndMeth=Zero  SaturateOnIntegerOverflow=on
  Gain : Gain  Gain=q0
  Gain1 : Gain  Gain=q1
  Gain2 : Gain  Gain=q2
  Integrator : Integrator
  Integrator1 : Integrator
  Integrator2 : Integrator
  Sum1 : Sum  Inputs=+-
  Sum2 : Sum  Inputs=----
  Sum3 : Sum  Inputs=+-
  Tanh : Trigonometry  Operator=tanh
  w : Constant  Value=w
  D3 : Outport  VectorParamsAs1DForOutWhenUnconnected=off
  wires:
  xd6/1 -> Sum1/2
  xd5/1 -> Sum3/2
  x5/1 -> Sum3/1
  x6/1 -> Sum1/1
  S6/1 -> [S6], Abs/1
  Sum1/1 -> [e2]
  Sum3/1 -> [e1]
  Gain/1 -> Integrator/1
  Integrator/1 -> Sum2/1  "B0"
  [e1] -> Divide/2
  Gain1/1 -> Integrator1/1
  Divide/1 -> Gain1/1
  Divide1/1 -> Gain2/1
  Gain2/1 -> Integrator2/1
  [e2] -> Divide1/2
  Abs/1 -> Divide1/1, Divide/1, Gain/1
  Integrator1/1 -> Divide3/2  "B1"
  w/1 -> Sum2/4
  Tanh/1 -> Divide2/2
  [S6] -> Tanh/1
  Divide2/1 -> D3/1
  [e1] -> Divide3/1
  [e2] -> Divide4/1
  Integrator2/1 -> Divide4/2  "B2"
  Divide3/1 -> Sum2/2
  Divide4/1 -> Sum2/3
  Sum2/1 -> Divide2/1

== system RobustFormationControl_FractionalModel/Fractional Leader with four followers/Follower 4 System/Follower 2 Quadrotor Model/Control Module1/Subsystem6/Subsystem3 ==
  xL : Inport
  x7 : Inport  Port=2
  x8 : Inport  Port=3
  dX : Inport  Port=4
  S8 : Inport  Port=5
  Constant : Constant  Value=p/q
  Constant1 : Constant  Value=gx-1
  Derivative : Derivative
  Derivative1 : Derivative
  Divide : Product  Inputs=**  RndMeth=Zero  SaturateOnIntegerOverflow=on
  Fractional derivative : fod/Fractional derivative  gam=alpha1(1)  ww=[0.001; 1000]  n=5  nFod=off
      settings: SourceProductName=FOMCON Toolbox
  Fractional integrator1 : fod/Fractional integrator  gam=alpha2(1)  ww=[0.001; 1000]  n=5  nFod=off
      settings: SourceProductName=FOMCON Toolbox
  Gain : Gain  Gain=cx1
  Gain1 : Gain  Gain=cx2
  Gain2 : Gain  Gain=gx
  Gain3 : Gain  Gain=Sigma1X
  Gain4 : Gain  Gain=Sigma2X
  Power : Math  Operator=pow
  Power1 : Math  Operator=pow
  Sum : Sum
  Sum1 : Sum  Inputs=+--
  Sum2 : Sum  Inputs=+++
  Sum3 : Sum  Inputs=+--
  Tanh : Trigonometry  Operator=tanh
  D2 : Outport  VectorParamsAs1DForOutWhenUnconnected=off
  wires:
  Sum3/1 -> Power1/1, Power/1
  Constant/1 -> Power/2
  Power/1 -> Gain/1
  Gain/1 -> Fractional derivative/1
  Constant1/1 -> Power1/2
  Power1/1 -> Divide/2
  Divide/1 -> Gain1/1
  Gain1/1 -> Gain2/1
  Sum1/1 -> Divide/1
  Gain2/1 -> Fractional integrator1/1
  S8/1 -> Tanh/1, Gain4/1
  Tanh/1 -> Gain3/1
  Gain3/1 -> Sum/1
  Gain4/1 -> Sum/2
  Sum/1 -> Sum2/3
  Fractional derivative/1 -> Sum2/1
  Fractional integrator1/1 -> Sum2/2
  Sum2/1 -> D2/1
  xL/1 -> Sum3/1, Derivative/1
  Derivative/1 -> Sum1/1
  x8/1 -> Sum1/2
  dX/1 -> Sum3/3, Derivative1/1
  Derivative1/1 -> Sum1/3
  x7/1 -> Sum3/2

== system RobustFormationControl_FractionalModel/Fractional Leader with four followers/Follower 4 System/Follower 2 Quadrotor Model/Control Module1/Subsystem6/Subsystem4 ==
  x8 : Inport
  xL : Inport  Port=2
  dX : Inport  Port=3
  Derivative{,1..3} (4 alike) : Derivative
  Divide2 : Product  Inputs=**  RndMeth=Zero  SaturateOnIntegerOverflow=on
  Gain1 : Gain  Commented=on  Gain=a6
  Sum : Sum  Inputs=-+-
  D1 : Outport
  wires:
  Sum/1 -> D1/1
  x8/1 -> Divide2/2
  Divide2/1 -> Sum/1
  [a4D] -> Divide2/1
  Derivative/1 -> Derivative1/1
  xL/1 -> Derivative/1
  Derivative3/1 -> Sum/3
  Derivative2/1 -> Derivative3/1
  dX/1 -> Derivative2/1
  Derivative1/1 -> Sum/2

== system RobustFormationControl_FractionalModel/Fractional Leader with four followers/Follower 4 System/Follower 2 Quadrotor Model/Control Module1/Subsystem6/Subsystem5 ==
  xL : Inport
  x7 : Inport  Port=2
  x8 : Inport  Port=3
  dX : Inport  Port=4
  S8 : Inport  Port=5
  Abs : Abs  SaturateOnIntegerOverflow=off
  Derivative : Derivative
  Derivative1 : Derivative
  Divide{,1..4} (5 alike) : Product  Inputs=**  RndMeth=Zero  SaturateOnIntegerOverflow=on
  Gain : Gain  Gain=q0
  Gain1 : Gain  Gain=q1
  Gain2 : Gain  Gain=q2
  Integrator : Integrator
  Integrator1 : Integrator
  Integrator2 : Integrator
  Sum2 : Sum  Inputs=++++
  Sum4 : Sum  Inputs=+--
  Sum5 : Sum  Inputs=+--
  Tanh : Trigonometry  Operator=tanh
  w : Constant  Value=w
  D3 : Outport  VectorParamsAs1DForOutWhenUnconnected=off
  wires:
  S8/1 -> [S8], Abs/1
  Gain/1 -> Integrator/1
  Integrator/1 -> Sum2/1  "B0"
  [e1] -> Divide/2
  Gain1/1 -> Integrator1/1
  Divide/1 -> Gain1/1
  Divide1/1 -> Gain2/1
  Gain2/1 -> Integrator2/1
  [e2] -> Divide1/2
  Abs/1 -> Divide1/1, Divide/1, Gain/1
  Integrator1/1 -> Divide3/2  "B1"
  w/1 -> Sum2/4
  Tanh/1 -> Divide2/2
  [S8] -> Tanh/1
  Divide2/1 -> D3/1
  [e1] -> Divide3/1
  [e2] -> Divide4/1
  Integrator2/1 -> Divide4/2  "B2"
  Divide3/1 -> Sum2/2
  Divide4/1 -> Sum2/3
  Sum2/1 -> Divide2/1
  Derivative1/1 -> Sum4/3
  Derivative/1 -> Sum4/1
  Sum4/1 -> [e2]
  Sum5/1 -> [e1]
  xL/1 -> Sum5/1, Derivative/1
  x8/1 -> Sum4/2
  dX/1 -> Sum5/3, Derivative1/1
  x7/1 -> Sum5/2

== system RobustFormationControl_FractionalModel/Fractional Leader with four followers/Follower 4 System/Follower 2 Quadrotor Model/Control Module1/Subsystem8/Subsystem ==
  x3 : Inport
  xd3 : Inport  Port=2
  x4 : Inport  Port=3
  xd4 : Inport  Port=4
  S4 : Inport  Port=5
  Constant : Constant  Value=p/q
  Constant1 : Constant  Value=gammaP(2)-1
  Divide : Product  Inputs=**  RndMeth=Zero  SaturateOnIntegerOverflow=on
  Fractional derivative : fod/Fractional derivative  gam=alpha1(2)  ww=[0.001; 1000]  n=5  nFod=off
      settings: SourceProductName=FOMCON Toolbox
  Fractional integrator1 : fod/Fractional integrator  gam=alpha2(2)  ww=[0.001; 1000]  n=5  nFod=off
      settings: SourceProductName=FOMCON Toolbox
  Gain : Gain  Gain=cTheta1
  Gain1 : Gain  Gain=cTheta2
  Gain2 : Gain  Gain=gammaP(2)
  Gain3 : Gain  Gain=Sigma1Theta
  Gain4 : Gain  Gain=Sigma2Theta
  Power : Math  Operator=pow
  Power1 : Math  Operator=pow
  Sum : Sum
  Sum1 : Sum  Inputs=+-
  Sum2 : Sum  Inputs=---
  Sum3 : Sum  Inputs=+-
  Tanh : Trigonometry  Operator=tanh
  D2 : Outport  VectorParamsAs1DForOutWhenUnconnected=off
  wires:
  xd4/1 -> Sum1/2
  xd3/1 -> Sum3/2
  x3/1 -> Sum3/1
  x4/1 -> Sum1/1
  Sum3/1 -> Power1/1, Power/1
  Constant/1 -> Power/2
  Power/1 -> Gain/1
  Gain/1 -> Fractional derivative/1
  Constant1/1 -> Power1/2
  Power1/1 -> Divide/2
  Divide/1 -> Gain1/1
  Gain1/1 -> Gain2/1
  Sum1/1 -> Divide/1
  Gain2/1 -> Fractional integrator1/1
  S4/1 -> Tanh/1, Gain4/1
  Tanh/1 -> Gain3/1
  Gain3/1 -> Sum/1
  Gain4/1 -> Sum/2
  Sum/1 -> Sum2/3
  Fractional derivative/1 -> Sum2/1
  Fractional integrator1/1 -> Sum2/2
  Sum2/1 -> D2/1

== system RobustFormationControl_FractionalModel/Fractional Leader with four followers/Follower 4 System/Follower 2 Quadrotor Model/Control Module1/Subsystem8/Subsystem1 ==
  x4 : Inport
  x6 : Inport  Port=2
  x2 : Inport  Port=3
  Omega : Inport  Port=4
  xd4 : Inport  Port=5
  Gain1 : Gain  Gain=a2
  Gain2 : Gain  Gain=c2
  Gain3 : Gain  Gain=b2
  Math Function1 : Math  Operator=square  SignedPower=on
  Product2 : Product
  Product4 : Product
  Sum3 : Sum  Inputs=---+
  D1 : Outport
  wires:
  x6/1 -> Product2/2
  Gain1/1 -> Sum3/1  "a1 x4 x6"
  Sum3/1 -> D1/1
  Math Function1/1 -> Gain2/1  "x2^2"
  x2/1 -> Product4/1, Product2/1
  x4/1 -> Math Function1/1
  xd4/1 -> Sum3/4
  Product4/1 -> Gain3/1
  Omega/1 -> Product4/2
  Product2/1 -> Gain1/1
  Gain3/1 -> Sum3/3
  Gain2/1 -> Sum3/2  "c1 x2^2"

== system RobustFormationControl_FractionalModel/Fractional Leader with four followers/Follower 4 System/Follower 2 Quadrotor Model/Control Module1/Subsystem8/Subsystem2 ==
  x3 : Inport
  xd3 : Inport  Port=2
  x4 : Inport  Port=3
  xd4 : Inport  Port=4
  S4 : Inport  Port=5
  Abs : Abs  SaturateOnIntegerOverflow=off
  Divide{,1..4} (5 alike) : Product  Inputs=**  RndMeth=Zero  SaturateOnIntegerOverflow=on
  Gain : Gain  Gain=q0
  Gain1 : Gain  Gain=q1
  Gain2 : Gain  Gain=q2
  Integrator : Integrator
  Integrator1 : Integrator
  Integrator2 : Integrator
  Sum1 : Sum  Inputs=+-
  Sum2 : Sum  Inputs=----
  Sum3 : Sum  Inputs=+-
  Tanh : Trigonometry  Operator=tanh
  w : Constant  Value=w
  D3 : Outport  VectorParamsAs1DForOutWhenUnconnected=off
  wires:
  xd4/1 -> Sum1/2
  xd3/1 -> Sum3/2
  x3/1 -> Sum3/1
  x4/1 -> Sum1/1
  S4/1 -> [S4], Abs/1
  Sum1/1 -> [e2]
  Sum3/1 -> [e1]
  Gain/1 -> Integrator/1
  Integrator/1 -> Sum2/1  "B0"
  [e1] -> Divide/2
  Gain1/1 -> Integrator1/1
  Divide/1 -> Gain1/1
  Divide1/1 -> Gain2/1
  Gain2/1 -> Integrator2/1
  [e2] -> Divide1/2
  Abs/1 -> Divide1/1, Divide/1, Gain/1
  Integrator1/1 -> Divide3/2  "B1"
  w/1 -> Sum2/4
  Tanh/1 -> Divide2/2
  [S4] -> Tanh/1
  Divide2/1 -> D3/1
  [e1] -> Divide3/1
  [e2] -> Divide4/1
  Integrator2/1 -> Divide4/2  "B2"
  Divide3/1 -> Sum2/2
  Divide4/1 -> Sum2/3
  Sum2/1 -> Divide2/1

== system RobustFormationControl_FractionalModel/Fractional Leader with four followers/Follower 4 System/Follower 2 Quadrotor Model/Quadrotor Dynamic System/Rotational System/Equation1 ==
  x4 : Inport
  x6 : Inport  Port=2
  U2 : Inport  Port=3
  Omega : Inport  Port=4
  Gain : Gain  Gain=a1
  Gain1 : Gain  Gain=c1
  Gain2 : Gain  Gain=b1
  Gain3 : Gain  Gain=d1
  Integrator : Integrator
  Integrator1 : Integrator
  Math Function : Math  Operator=square  SignedPower=on
  Product : Product
  Product1 : Product
  Sum : Sum  Inputs=|++++
  x1 = Phi : Outport  VectorParamsAs1DForOutWhenUnconnected=off
  x2 : Outport  Port=2  VectorParamsAs1DForOutWhenUnconnected=off
  wires:
  Math Function/1 -> Gain1/1  "x2^2"
  x4/1 -> Product1/1, Product/1
  Integrator/1 -> Math Function/1, x2/1, Integrator1/1
  U2/1 -> Gain3/1
  Gain2/1 -> Sum/3
  Gain3/1 -> Sum/4
  Gain/1 -> Sum/1  "a1 x4 x6"
  Product1/1 -> Gain2/1
  Gain1/1 -> Sum/2  "c1 x2^2"
  Integrator1/1 -> x1 = Phi/1
  Product/1 -> Gain/1
  x6/1 -> Product/2
  Sum/1 -> Integrator/1
  Omega/1 -> Product1/2
